simulink model "PV_GFL_864_SystemLevel_SM_R2"  (R2026a)
settings: Solver=ode23t  StopTime=0.20  MaxStep=1e-5
InitFcn:
  | run(fullfile(fileparts(get_param(bdroot,'FileName')),'..','scripts','init_pv_gfl_864_average_sm.m'));
undefined symbols (not defined in the file): Control, DiscIntNeverNeededParam, ee, GridTransformer, S1, SM, Ts
libraries: ee_lib x17, nesl_utility x15, fl_lib x5, simulink x1, eeSmAC1C x1
Description:
  | B2 readable SRF-PLL, dq measurement, and P/Q estimation on the validated B1 switching plant.
settings Model: Creator=fakebob2004  LastModifiedBy=fakebob2004

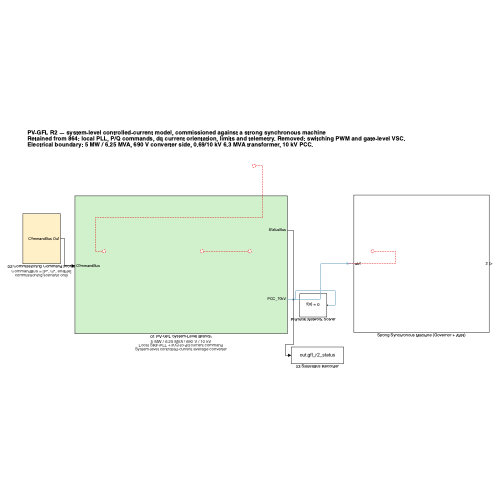
[thumbnail: Simulink's stored preview of the top-level diagram]
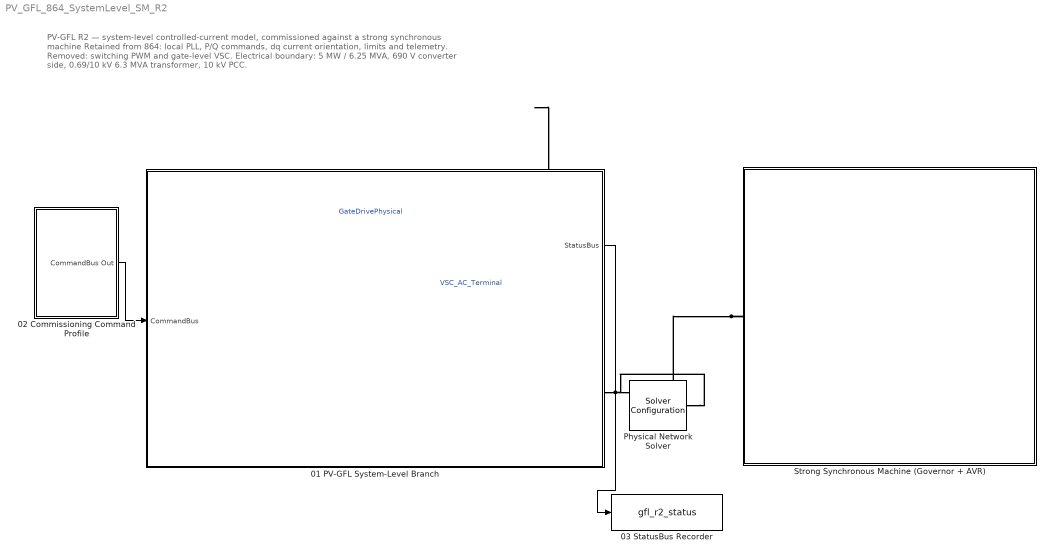
== system PV_GFL_864_SystemLevel_SM_R2 ==
  note: PV-GFL R2 — system-level controlled-current model, commissioned against a strong synchronous machine
      | Retained from 864: local PLL, P/Q commands, dq current orientation, limits and telemetry. Removed: switching PWM and gate-level VSC.
      | Electrical boundary: 5 MW / 6.25 MVA, 690 V converter side, 0.69/10 kV 6.3 MVA transformer, 10 kV PCC.
  01 PV-GFL System-Level Branch : Subsystem
      settings: AttributesFormatString=|
      | 5 MW / 6.25 MVA | 690 V / 10 kV
      | Local SRF-PLL + P/Q-to-dq current command
      | System-level controlled-current average converter
  02 Commissioning Command Profile : Subsystem
      settings: AttributesFormatString=|
      | CommandBus = [P*, Q*, enable]
      | commissioning scenario only
  03 StatusBus Recorder : ToWorkspace  VariableName=gfl_r2_status  SampleTime=-1
  Physical Network Solver : nesl_utility/Solver Configuration  PhysicalDomain=network_engine_domain  SubClassName=solver  LeftPortType=input  RightPortType=generic  Tones=[]  Harmonics=[]  SimulateNoise=off  Profile=off  UseLocalSampling=off  EnableSwitchedLinearOptims=on  FrequencyDomain=off  UseCCode=off  RelTol=0.001  AbsTol=0.001  MinStep=1e-09  ToWorkspace=off  RevertToSquareIcSolve=off  NumHomotopyIterations=100  PhasorMode=off  PhasorModeNumHarmonics=1  ConsistencySolver=NEWTON_XTOL_AFTER_FTOL  CanonicalOrdering=CANONICAL  OptimizeIntermediates=OPTIMIZED  IndexReductionMethod=DerivativeReplacement  DoDC=off  ResidualTolerance=1e-09  ConsistencyTolSource=GLOBAL  ConsistencyAbsTol=0.001  ConsistencyRelTol=0.001  ConsistencyTolFactor=0.001  UseLocalSolver=off  LocalSolverChoice=NE_BACKWARD_EULER_ADVANCER  ResolveIndetEquations=on  FunctionEvalNumThread=1  LocalSolverSampleTime=0.001  DoFixedCost=off  MaxNonlinIter=3  MaxModeIter=2  ComputeImpulses=off  ImpulseIterations=2  LinearAlgebra=auto  LinearAlgebraNumThread=0  EquationFormulation=NE_TIME_EF  DelaysMemoryBudget=1024  AutomaticFiltering=on  FilteringTimeConstant=0.001  PartitionStorageMethod=AS_NEEDED  PartitionMemoryBudget=1024  PartitionMethod=ROBUST  MultibodyUseLocalSolver=off  MultibodyLocalSolverChoice=ODE1  MultibodyLocalSolverSampleTime=0.001
  Strong Synchronous Machine (Governor + AVR) : Subsystem  VariantControl=SynchronousMachine
  wires:
  02 Commissioning Command Profile/1(CommandBus Out) -> 01 PV-GFL System-Level Branch/1(CommandBus)
  01 PV-GFL System-Level Branch/1(StatusBus) -> 03 StatusBus Recorder/1
  connections:
  ?  "VSC_AC_Terminal"
  ?  "GateDrivePhysical"
  Strong Synchronous Machine (Governor + AVR)/RConn1 -- 01 PV-GFL System-Level Branch/RConn1 -- Physical Network Solver/RConn1

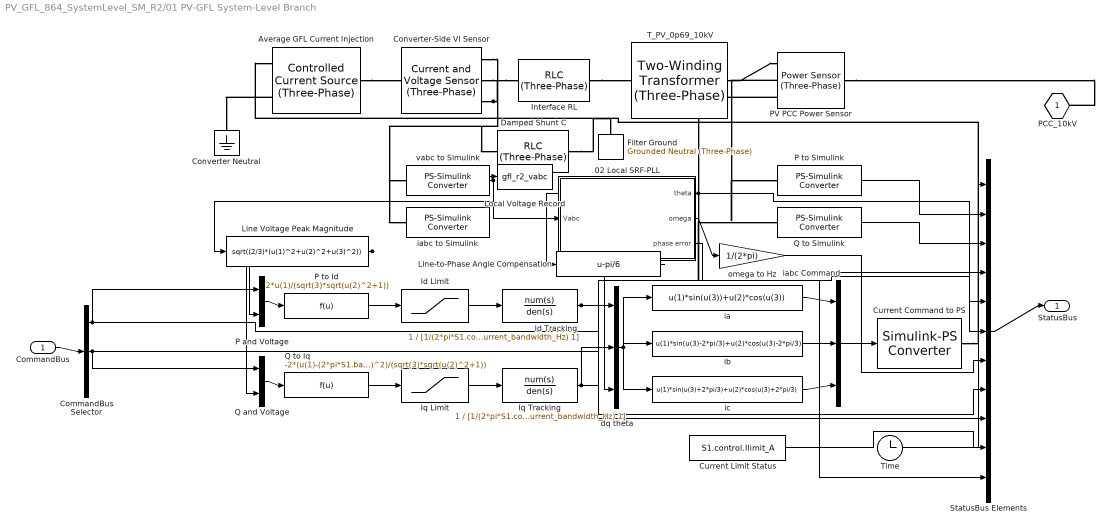
== system PV_GFL_864_SystemLevel_SM_R2/01 PV-GFL System-Level Branch ==
  CommandBus : Inport
  02 Local SRF-PLL : Subsystem
      settings: AttributesFormatString=|
      | local abc voltage only
      | wrapped phase-error PI
  Average GFL Current Injection : ee_lib/Sources/Controlled Current Source (Three-Phase)  port_option=ee.enum.threePhasePort.composite  input_option=ee.enum.inputType.instantaneous  FRated=S1.base.f_Hz Hz  G_parasitic=0 1/Ohm
  CommandBus Selector : Demux  Outputs=3
  Converter Neutral : fl_lib/Electrical/Electrical Elements/Electrical Reference
  Converter-Side VI Sensor : ee_lib/Sensors & Transducers/Current and Voltage Sensor (Three-Phase)  port_option=ee.enum.threePhasePort.composite  vMeasurementType=ee.enum.vmeasurement.ll  outputUnit=ee.enum.unit.si  SRated=100e6 A*V  VRated=24e3 V  I_specify=off  I_priority=None  I=[0, 0, 0] A  I_nominal_specify=off  I_nominal_value=1  I_nominal_unit=A  V_specify=off  V_priority=None  V=[0, 0, 0] V  V_nominal_specify=off  V_nominal_value=1  V_nominal_unit=V
  Current Command to PS : nesl_utility/Simulink-PS Converter  PhysicalDomain=network_engine_domain  SubClassName=ps_input  LeftPortType=input  RightPortType=output  PseudoPeriodic=off  Frequencies=[]  NoiseDistribution=none  NoiseParameters=[]  Unit=A  AffineConversion=off  FilteringAndDerivatives=zero  SimscapeFilterOrder=1  InputFilterTimeConstant=0.001  UdotUserProvided=0
  Current Limit Status : Constant  Value=S1.control.Ilimit_A
  Damped Shunt C : ee_lib/Passive/RLC Assemblies/RLC (Three-Phase)  port_option=ee.enum.threePhasePort.composite  component_structure=ee.enum.rlc.structure.SeriesRC  R=S1.filter.Rd_ohm Ohm  L=1e-3 H  C=S1.filter.C_F F  R_parasitic=0 Ohm  G_parasitic=0 1/Ohm  IL_specify=off  IL_priority=High  IL=[0, 0, 0] A  IL_nominal_specify=off  IL_nominal_value=1  IL_nominal_unit=A  VC_specify=off  VC_priority=High  VC=[0, 0, 0] V  VC_nominal_specify=off  VC_nominal_value=1  VC_nominal_unit=V
  Filter Ground : ee_lib/Connectors & References/Grounded Neutral (Three-Phase)  port_option=ee.enum.threePhasePort.composite
  Id Limit : Saturate  UpperLimit=S1.control.Ilimit_A  LowerLimit=-S1.control.Ilimit_A
  Id Tracking : TransferFcn  Numerator=1  Denominator=[1/(2*pi*S1.control.current_bandwidth_Hz) 1]
  Interface RL : ee_lib/Passive/RLC Assemblies/RLC (Three-Phase)  port_option=ee.enum.threePhasePort.composite  component_structure=ee.enum.rlc.structure.R  R=S1.filter.R1_ohm+S1.filter.R2_ohm Ohm  L=1e-3 H  C=1e-6 F  R_parasitic=0 Ohm  G_parasitic=0 1/Ohm  IL_specify=off  IL_priority=High  IL=[0, 0, 0] A  IL_nominal_specify=off  IL_nominal_value=1  IL_nominal_unit=A  VC_specify=off  VC_priority=High  VC=[0, 0, 0] V  VC_nominal_specify=off  VC_nominal_value=1  VC_nominal_unit=V
  Iq Limit : Saturate  UpperLimit=S1.control.Ilimit_A  LowerLimit=-S1.control.Ilimit_A
  Iq Tracking : TransferFcn  Numerator=1  Denominator=[1/(2*pi*S1.control.current_bandwidth_Hz) 1]
  Line Voltage Peak Magnitude : Fcn  Expr=sqrt((2/3)*(u(1)^2+u(2)^2+u(3)^2))
  Line-to-Phase Angle Compensation : Fcn  Expr=u-pi/6
  Local Voltage Record : ToWorkspace  VariableName=gfl_r2_vabc  SampleTime=-1
  P and Voltage : Mux  Inputs=2
  P to Id : Fcn  Expr=2*u(1)/(sqrt(3)*sqrt(u(2)^2+1))
  P to Simulink : nesl_utility/PS-Simulink Converter  PhysicalDomain=network_engine_domain  SubClassName=ps_output  LeftPortType=input  RightPortType=output  PseudoPeriodic=off  Frequencies=[]  VectorFormat=inherit  Unit=W  AffineConversion=off
  PV PCC Power Sensor : ee_lib/Sensors & Transducers/Power Sensor (Three-Phase)  port_option=ee.enum.threePhasePort.composite  load_type=ee.enum.passive.type_balanced.balanced  f0=60 Hz
  Q and Voltage : Mux  Inputs=2
  Q to Iq : Fcn  Expr=-2*(u(1)-(2*pi*S1.base.f_Hz*S1.filter.C_F/2)*u(2)^2)/(sqrt(3)*sqrt(u(2)^2+1))
  Q to Simulink : nesl_utility/PS-Simulink Converter  PhysicalDomain=network_engine_domain  SubClassName=ps_output  LeftPortType=input  RightPortType=output  PseudoPeriodic=off  Frequencies=[]  VectorFormat=inherit  Unit=W  AffineConversion=off
  StatusBus Elements : Mux  Inputs=11
  T_PV_0p69_10kV : ee_lib/Passive/Transformers/Two-Winding Transformer (Three-Phase)  SRated=S1.transformer.S_VA A*V  FRated=S1.base.f_Hz Hz  Winding1Connection=ee.enum.windingconnection.Yg  VRated1=S1.pv.Vll_low_V V  Winding2Connection=ee.enum.windingconnection.Yg  VRated2=S1.pv.Vll_high_V V  CoreType=ee.enum.coretype.threelimb  pu_Rw1=S1.transformer.R_pu/2  pu_Rw2=S1.transformer.R_pu/2  leakage_reactance_option=ee.enum.transformer_leakage.exclude  pu_Xl1=0.05  pu_Xl2=0.05  magnetizing_resistance_option=ee.enum.transformer_magnetizingResistance.exclude  pu_Rm=500  magnetizing_reactance_option=ee.enum.transformer_magnetizingReactance.exclude  saturation_option=ee.enum.transformer_saturation.exclude  pu_Xm=500  current_data=[0, .002, 1, 2]  magnetic_flux_data=[0, 1.2, 1.5, 1.51]  pu_X0=0.5  i1_specify=off  i1_priority=None  i1=[0, 0, 0] A  i1_nominal_specify=off  i1_nominal_value=1  i1_nominal_unit=A  i2_specify=off  i2_priority=None  i2=[0, 0, 0] A  i2_nominal_specify=off  i2_nominal_value=1  i2_nominal_unit=A  phi_specify=off  phi_priority=None  phi=[0, 0, 0]  phi_nominal_specify=off  phi_nominal_value=1  phi_nominal_unit=1
  Time : Clock
  dq theta : Mux  Inputs=3
  ia : Fcn  Expr=u(1)*sin(u(3))+u(2)*cos(u(3))
  iabc Command : Mux  Inputs=3
  iabc to Simulink : nesl_utility/PS-Simulink Converter  PhysicalDomain=network_engine_domain  SubClassName=ps_output  LeftPortType=input  RightPortType=output  PseudoPeriodic=off  Frequencies=[]  VectorFormat=inherit  Unit=A  AffineConversion=off
  ib : Fcn  Expr=u(1)*sin(u(3)-2*pi/3)+u(2)*cos(u(3)-2*pi/3)
  ic : Fcn  Expr=u(1)*sin(u(3)+2*pi/3)+u(2)*cos(u(3)+2*pi/3)
  omega to Hz : Gain  Gain=1/(2*pi)
  vabc to Simulink : nesl_utility/PS-Simulink Converter  PhysicalDomain=network_engine_domain  SubClassName=ps_output  LeftPortType=input  RightPortType=output  PseudoPeriodic=off  Frequencies=[]  VectorFormat=inherit  Unit=V  AffineConversion=off
  PCC_10kV : PMIOPort  Side=Right  ConnectionType=Connection: foundation.electrical.three_phase
  StatusBus : Outport
  wires:
  CommandBus/1 -> CommandBus Selector/1
  vabc to Simulink/1 -> Local Voltage Record/1, 02 Local SRF-PLL/1(Vabc), Line Voltage Peak Magnitude/1
  CommandBus Selector/1 -> P and Voltage/1, StatusBus Elements/4
  Line Voltage Peak Magnitude/1 -> P and Voltage/2, Q and Voltage/2
  CommandBus Selector/2 -> Q and Voltage/1, StatusBus Elements/5
  P and Voltage/1 -> P to Id/1
  P to Id/1 -> Id Limit/1
  Id Limit/1 -> Id Tracking/1
  Q and Voltage/1 -> Q to Iq/1
  Q to Iq/1 -> Iq Limit/1
  Iq Limit/1 -> Iq Tracking/1
  Id Tracking/1 -> dq theta/1, StatusBus Elements/8
  Iq Tracking/1 -> dq theta/2, StatusBus Elements/9
  02 Local SRF-PLL/1(theta) -> Line-to-Phase Angle Compensation/1, StatusBus Elements/6
  Line-to-Phase Angle Compensation/1 -> dq theta/3
  dq theta/1 -> ia/1, ib/1, ic/1
  ia/1 -> iabc Command/1
  ib/1 -> iabc Command/2
  ic/1 -> iabc Command/3
  iabc Command/1 -> Current Command to PS/1
  02 Local SRF-PLL/2(omega) -> omega to Hz/1
  Time/1 -> StatusBus Elements/1
  P to Simulink/1 -> StatusBus Elements/2
  Q to Simulink/1 -> StatusBus Elements/3
  omega to Hz/1 -> StatusBus Elements/7
  Current Limit Status/1 -> StatusBus Elements/10
  02 Local SRF-PLL/3(phase error) -> StatusBus Elements/11
  StatusBus Elements/1 -> StatusBus/1
  connections:
  Average GFL Current Injection/LConn2 -- Converter Neutral/LConn1
  Average GFL Current Injection/RConn1 -- Converter-Side VI Sensor/LConn1
  Interface RL/LConn1 -- Converter-Side VI Sensor/RConn3 -- Damped Shunt C/LConn1
  Damped Shunt C/RConn1 -- Filter Ground/LConn1
  Interface RL/RConn1 -- T_PV_0p69_10kV/LConn1
  T_PV_0p69_10kV/RConn1 -- PV PCC Power Sensor/LConn1
  PV PCC Power Sensor/RConn1 -- PCC_10kV/RConn1
  Converter-Side VI Sensor/RConn1 -- vabc to Simulink/LConn1
  Converter-Side VI Sensor/RConn2 -- iabc to Simulink/LConn1
  PV PCC Power Sensor/LConn2 -- P to Simulink/LConn1
  PV PCC Power Sensor/LConn3 -- Q to Simulink/LConn1
  Current Command to PS/RConn1 -- Average GFL Current Injection/LConn1

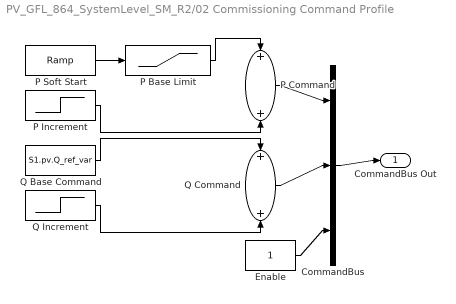
== system PV_GFL_864_SystemLevel_SM_R2/02 Commissioning Command Profile ==
  CommandBus : Mux  Inputs=3
  Enable : Constant
  P Base Limit : Saturate  UpperLimit=S1.pv.P_initial_W  LowerLimit=0
  P Command : Sum
  P Increment : Step  Time=S1.pv.P_step_time_s  FinalValue=S1.pv.P_final_W-S1.pv.P_initial_W  SampleTime=0
  P Soft Start : simulink/Sources/Ramp  slope=S1.pv.P_ramp_W_per_s  start=0  InitialOutput=0
  Q Base Command : Constant  Value=S1.pv.Q_ref_var
  Q Command : Sum
  Q Increment : Step  Time=S1.pv.Q_step_time_s  FinalValue=S1.pv.Q_step_var  SampleTime=0
  CommandBus Out : Outport
  wires:
  P Soft Start/1 -> P Base Limit/1
  P Base Limit/1 -> P Command/1
  P Increment/1 -> P Command/2
  Q Base Command/1 -> Q Command/1
  Q Increment/1 -> Q Command/2
  P Command/1 -> CommandBus/1
  Q Command/1 -> CommandBus/2
  Enable/1 -> CommandBus/3
  CommandBus/1 -> CommandBus Out/1

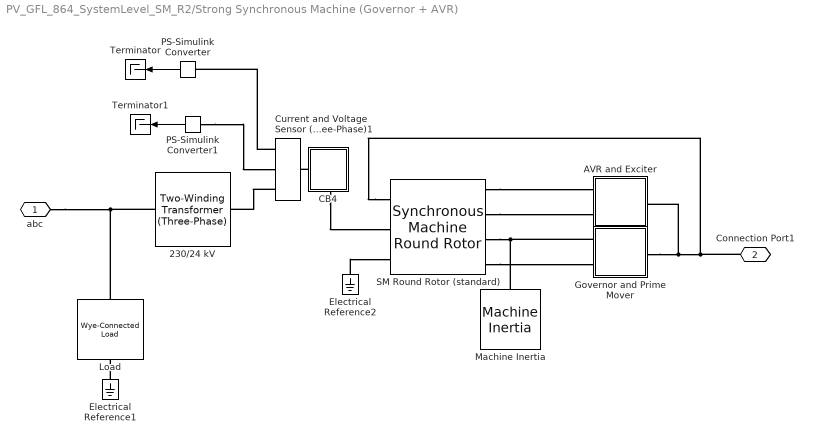
== system PV_GFL_864_SystemLevel_SM_R2/Strong Synchronous Machine (Governor + AVR) ==
  " Load" : ee_lib/Passive/RLC Assemblies/Wye-Connected Load  port_option=ee.enum.threePhasePort.composite  parameterization=ee.enum.rlc.parameterization.ratedpower  component_structure=ee.enum.rlc.structure.R  component_structure_PQ=ee.enum.rlc.structure.ParallelRL  R=1 Ohm  L=1e-3 H  C=1e-6 F  VRated=Grid.voltage V  FRated=Grid.frequency Hz  P=SM.P_load W  Qpos=SM.Q_load A*V  Qneg=-1e2 A*V  R_parasitic=0 Ohm  G_parasitic=0 1/Ohm  R_parasitic_PQ=0 Ohm  G_parasitic_PQ=0 1/Ohm  Vmag0=4.16e3 V  Vang0=0 deg  Freq0=60 Hz  IL_specify=off  IL_priority=High  IL=[0, 0, 0] A  IL_nominal_specify=off  IL_nominal_value=1  IL_nominal_unit=A  VC_specify=off  VC_priority=High  VC=[0, 0, 0] V  VC_nominal_specify=off  VC_nominal_value=1  VC_nominal_unit=V
  230/24 kV : ee_lib/Passive/Transformers/Two-Winding Transformer (Three-Phase)  SRated=SM.MVA V*A  FRated=Grid.frequency Hz  Winding1Connection=ee.enum.windingconnection.delta1  VRated1=Grid.voltage V  Winding2Connection=ee.enum.windingconnection.delta11  VRated2=SM.Voltage V  CoreType=ee.enum.coretype.fivelimb  pu_Rw1=GridTransformer.winding_resistance/2  pu_Rw2=GridTransformer.winding_resistance/2  leakage_reactance_option=ee.enum.transformer_leakage.include  pu_Xl1=GridTransformer.winding_lekage_reactance/2  pu_Xl2=GridTransformer.winding_lekage_reactance/2  magnetizing_resistance_option=ee.enum.transformer_magnetizingResistance.exclude  pu_Rm=500  magnetizing_reactance_option=ee.enum.transformer_magnetizingReactance.include  saturation_option=ee.enum.transformer_saturation.exclude  pu_Xm=500  current_data=[0, .002, 1, 2]  magnetic_flux_data=[0, 1.2, 1.5, 1.51]  pu_X0=0.0586/2  i1_specify=off  i1_priority=None  i1=[ 0 0 0 ] A  i1_nominal_specify=off  i1_nominal_value=1  i1_nominal_unit=A  i2_specify=off  i2_priority=None  i2=[ 0 0 0 ] A  i2_nominal_specify=off  i2_nominal_value=1  i2_nominal_unit=A  phi_specify=off  phi_priority=None  phi=[ 0 0 0 ]  phi_nominal_specify=off  phi_nominal_value=1  phi_nominal_unit=1
  AVR and Exciter : Subsystem
  CB4 : Subsystem
      settings: PortSchema="{\"entries\":[{\"content\":{\"sides\":[{\"content\":{\"connectorIds\":[\"LConn1\"]},\"type\":\"ConnectorPlacement.EquallySpacedRectSide\",\"uuid\":\"24022911-97b6-486c-a625-f0780a134feb\"},{\"content\":{\"connectorIds\":[],\"side\":\"RIGHT\"},\"type\":\"ConnectorPlacement.EquallySpacedRectSide\",\"uuid\":\"1242aa8b-343b-4af2-8b96-dfa58505a53d\"},{\"content\":{\"connectorIds\":[],\"side\":\"TOP\"},\"type\":\"ConnectorPlacement.EquallySpacedRectSide\",\"uuid\":\"e73be2e9-5300-480f-914f-665ff518f6ad\"},{\"content\":{\"connectorIds\":[\"RConn1\"],\"side\":\"BOTTOM\"},\"type\":\"ConnectorPlacement.EquallySpacedRectSide\",\"uuid\":\"6525202c-c4e7-4c96-9421-427b801d0594\"}]},\"type\":\"ConnectorPlacement.EquallySpacedConnector\",\"uuid\":\"b455682c-e951-4ef6-bff8-cd3f50b315f1\"}],\"packageUris\":[\"http://schema.mathworks.com/mf0/Connector/R2020b\"],\"version\":\"1.0\"}"
      mask Display: image('$imagefile'); % Use "Edit Image" on toolstrip to change.
  Current and Voltage Sensor (Three-Phase)1 : ee_lib/Sensors & Transducers/Current and Voltage Sensor (Three-Phase)  port_option=ee.enum.threePhasePort.composite  vMeasurementType=ee.enum.vmeasurement.ll  outputUnit=ee.enum.unit.pu  SRated=100e6 A*V  VRated=4.16e3 V  I_specify=off  I_priority=None  I=[0, 0, 0] A  I_nominal_specify=off  I_nominal_value=1  I_nominal_unit=A  V_specify=off  V_priority=None  V=[0, 0, 0] V  V_nominal_specify=off  V_nominal_value=1  V_nominal_unit=V
  Electrical Reference1 : fl_lib/Electrical/Electrical Elements/Electrical Reference
  Electrical Reference2 : fl_lib/Electrical/Electrical Elements/Electrical Reference
  "Governor and Prime Mover " : Subsystem  mask(Governor and Prime Mover){pu_speed_reference=SM.speed_reference, droop_percentage=SM.droop_p, pu_load_reference_setpoint=SM.load_reference_set_point, T_G=SM.governor_time_constant, T_CH=SM.time_constsnt_steamchest, base_torque=SM.Base_Torque_SM, pu_torque0=SM.initial_torque}
      mask prompts: pu_speed_reference "Speed reference, (pu)"; droop_percentage "Percentage droop, (%)"; pu_load_reference_setpoint "Load reference setpoint, (pu)"; T_G "Time constant of governor, (s)"; T_CH "Time constant of main inlet volumes and steam chest, (s)"; base_torque "Base torque, (N*m)"; pu_torque0 "Initial torque, (pu)"
      mask help:
      | Implements a synchronous machine governor and prime mover. The prime mover is a non-reheat steam turbine.
      |
      | The input to the block is a per-unit synchronous machine measurement vector.
      |
      | R and C are mechanical rotational ports.
  Machine Inertia : ee_lib/Electromechanical/Mechanical/Machine Inertia  SRated=SM.MVA V*A  FRated=Grid.frequency Hz  nPolePairs=SM.polepairs  inertia_option=2  J=27548 kg*m^2  H=SM.inertia s  damper_option=2  D=39.0509 N*m/(rad/s)  pu_D=SM.damping  initialization_option=2  fMechanical0=60 Hz  fElectrical0=Grid.frequency Hz
  PS-Simulink Converter : nesl_utility/PS-Simulink Converter  PhysicalDomain=network_engine_domain  SubClassName=ps_output  LeftPortType=input  RightPortType=output  PseudoPeriodic=off  Frequencies=[]  VectorFormat=inherit  Unit=inherit  AffineConversion=off
  PS-Simulink Converter1 : nesl_utility/PS-Simulink Converter  PhysicalDomain=network_engine_domain  SubClassName=ps_output  LeftPortType=input  RightPortType=output  PseudoPeriodic=off  Frequencies=[]  VectorFormat=inherit  Unit=inherit  AffineConversion=off
  SM Round Rotor (standard) : ee_lib/Electromechanical/Synchronous/Synchronous Machine Round Rotor  port_option=ee.enum.threePhasePort.composite  SRated=SM.MVA V*A  VRated=SM.Voltage V  FRated=Grid.frequency Hz  nPolePairs=SM.polepairs  param_option=ee.enum.sm.parameterization.standard  fieldCircuitParameterization_option=2  baseEfd=92.95 V  baseIfd=SM.field_current A  zero_sequence=ee.enum.park.zerosequence.include  axes_param=ee.enum.rotorangle.qaxis  Ladu=1.66  Laqu=1.61  L0=0.15  Ll=0.15  Ra=SM.stator_resistance  Lfd=0.165  Rfd=0.0006  L1d=0.1713  R1d=0.0284  L1q=0.7252  R1q=0.00619  L2q=0.125  R2q=0.02368  Xl=SM.lekage_reactance  Xd=SM.xd  Xq=SM.xq  X0=0.15  Xdd=SM.xd_  Xqd=SM.xq_  Xddd=SM.xd_dash  Xqdd=SM.xq_dash  d_option=1  Td0d=SM.Tdo_ s  Tdd=1.3260 s  Td0dd=SM.Tdo_dash s  Tddd=0.0230 s  q_option=1  Tq0d=SM.Tqo_ s  Tqd=0.3693 s  Tq0dd=SM.Tqo_dash s  Tqdd=0.0269 s  saturation_option=0  saturation_ifd=[0.00, 0.48, 0.76, 1.38, 1.79]  saturation_Vag=[0.00, 0.80, 1.08, 1.31, 1.40]  initialization_option=2  source_type=ee.enum.sm.load_flow_source_type.Swing  Vmag0=SM.Voltage V  Vang0=0 deg  Pt0=SM.initial_Pe V*A  Qt0=SM.initial_Qe V*A  minimum_pu=0.95  phase_search_range=[-inf, inf] deg  gmin=1e-6 S  connection_option=int32(ee.enum.Connection.wye)  num_q_dampers=2  rotor_offset=-pi / 2 rad  pu_psid_specify=on  pu_psid_priority=High  pu_psid=0  pu_psid_nominal_specify=off  pu_psid_nominal_value=1  pu_psid_nominal_unit=1  pu_psiq_specify=on  pu_psiq_priority=High  pu_psiq=0  pu_psiq_nominal_specify=off  pu_psiq_nominal_value=1  pu_psiq_nominal_unit=1  pu_psifd_specify=on  pu_psifd_priority=High  pu_psifd=0  pu_psifd_nominal_specify=off  pu_psifd_nominal_value=1  pu_psifd_nominal_unit=1  pu_psi1d_specify=on  pu_psi1d_priority=High  pu_psi1d=0  pu_psi1d_nominal_specify=off  pu_psi1d_nominal_value=1  pu_psi1d_nominal_unit=1  pu_psi1q_specify=on  pu_psi1q_priority=High  pu_psi1q=0  pu_psi1q_nominal_specify=off  pu_psi1q_nominal_value=1  pu_psi1q_nominal_unit=1  pu_psi2q_specify=on  pu_psi2q_priority=High  pu_psi2q=0  pu_psi2q_nominal_specify=off  pu_psi2q_nominal_value=1  pu_psi2q_nominal_unit=1  angular_position_diff_specify=on  angular_position_diff_priority=High  angular_position_diff=0 deg  angular_position_diff_nominal_specify=off  angular_position_diff_nominal_value=1  angular_position_diff_nominal_unit=deg  Tmeas=298.15 K  alpha=3.93e-3 1/K  stator_thermal_mass=100 J/K  rotor_thermal_mass=200 J/K  temperatureA_specify=off  temperatureA_priority=High  temperatureA=25 degC  temperatureA_nominal_specify=off  temperatureA_nominal_value=1  temperatureA_nominal_unit=degC  temperatureB_specify=off  temperatureB_priority=High  temperatureB=25 degC  temperatureB_nominal_specify=off  temperatureB_nominal_value=1  temperatureB_nominal_unit=degC  temperatureC_specify=off  temperatureC_priority=High  temperatureC=25 degC  temperatureC_nominal_specify=off  temperatureC_nominal_value=1  temperatureC_nominal_unit=degC  temperatureR_specify=off  temperatureR_priority=High  temperatureR=25 degC  temperatureR_nominal_specify=off  temperatureR_nominal_value=1  temperatureR_nominal_unit=degC
  Terminator : Terminator
  Terminator1 : Terminator
  abc : PMIOPort  Side=Right
  Connection Port1 : PMIOPort  Port=2  Side=Left
  wires:
  PS-Simulink Converter1/1 -> Terminator1/1
  PS-Simulink Converter/1 -> Terminator/1
  connections:
  Electrical Reference2/LConn1 -- SM Round Rotor (standard)/RConn3
  CB4/RConn1 -- SM Round Rotor (standard)/RConn2
  PS-Simulink Converter1/LConn1 -- Current and Voltage Sensor (Three-Phase)1/RConn2
  Current and Voltage Sensor (Three-Phase)1/RConn3 -- 230/24 kV/RConn1
  SM Round Rotor (standard)/LConn2 -- AVR and Exciter/RConn2
  Electrical Reference1/LConn1 -- " Load"/RConn1
  CB4/LConn1 -- Current and Voltage Sensor (Three-Phase)1/LConn1
  SM Round Rotor (standard)/LConn1 -- AVR and Exciter/RConn1
  Current and Voltage Sensor (Three-Phase)1/RConn1 -- PS-Simulink Converter/LConn1
  SM Round Rotor (standard)/LConn4 -- "Governor and Prime Mover "/RConn2
  "Governor and Prime Mover "/RConn1 -- Machine Inertia/LConn1 -- SM Round Rotor (standard)/LConn3
  SM Round Rotor (standard)/RConn1 -- Connection Port1/RConn1 -- AVR and Exciter/LConn1 -- "Governor and Prime Mover "/LConn1
  230/24 kV/LConn1 -- abc/RConn1 -- " Load"/LConn1

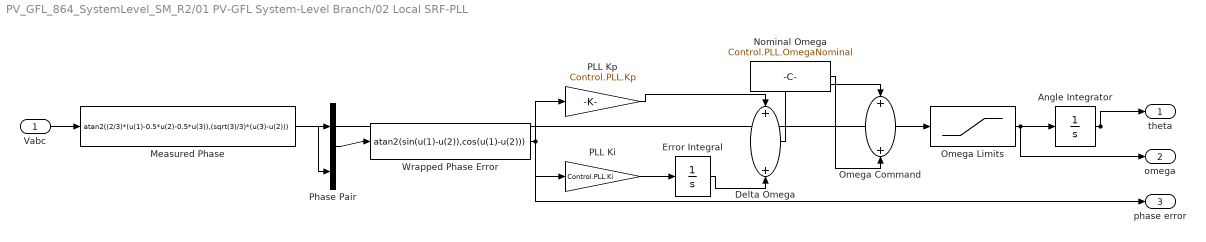
== system PV_GFL_864_SystemLevel_SM_R2/01 PV-GFL System-Level Branch/02 Local SRF-PLL ==
  Vabc : Inport
  Angle Integrator : Integrator  InitialCondition=Control.PLL.Theta0
  Delta Omega : Sum
  Error Integral : Integrator
  Measured Phase : Fcn  Expr=atan2((2/3)*(u(1)-0.5*u(2)-0.5*u(3)),(sqrt(3)/3)*(u(3)-u(2)))
  Nominal Omega : Constant  Value=Control.PLL.OmegaNominal
  Omega Command : Sum
  Omega Limits : Saturate  UpperLimit=Control.PLL.OmegaMax  LowerLimit=Control.PLL.OmegaMin
  PLL Ki : Gain  Gain=Control.PLL.Ki
  PLL Kp : Gain  Gain=Control.PLL.Kp
  Phase Pair : Mux  Inputs=2
  Wrapped Phase Error : Fcn  Expr=atan2(sin(u(1)-u(2)),cos(u(1)-u(2)))
  theta : Outport
  omega : Outport  Port=2
  phase error : Outport  Port=3
  wires:
  Vabc/1 -> Measured Phase/1
  Measured Phase/1 -> Phase Pair/1
  Angle Integrator/1 -> Phase Pair/2, theta/1
  Phase Pair/1 -> Wrapped Phase Error/1
  Wrapped Phase Error/1 -> PLL Kp/1, PLL Ki/1, phase error/1
  PLL Ki/1 -> Error Integral/1
  PLL Kp/1 -> Delta Omega/1
  Error Integral/1 -> Delta Omega/2
  Delta Omega/1 -> Omega Command/1
  Nominal Omega/1 -> Omega Command/2
  Omega Command/1 -> Omega Limits/1
  Omega Limits/1 -> Angle Integrator/1, omega/1

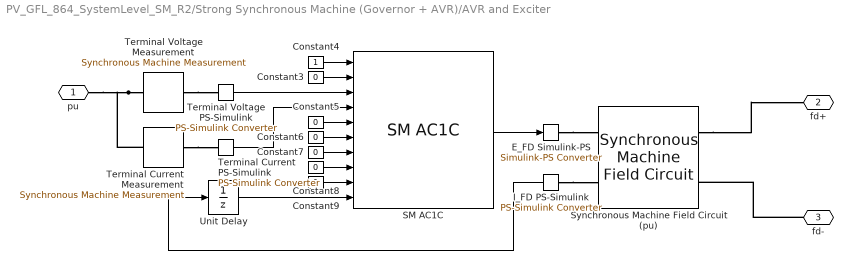
== system PV_GFL_864_SystemLevel_SM_R2/Strong Synchronous Machine (Governor + AVR)/AVR and Exciter ==
  Constant{3,5..9} (6 alike) : Constant  Value=0
  Constant4 : Constant
  "E_FD Simulink-PS " : nesl_utility/Simulink-PS Converter  PhysicalDomain=network_engine_domain  SubClassName=ps_input  LeftPortType=input  RightPortType=output  PseudoPeriodic=off  Frequencies=[]  NoiseDistribution=none  NoiseParameters=[]  Unit=1  AffineConversion=off  FilteringAndDerivatives=zero  SimscapeFilterOrder=1  InputFilterTimeConstant=.001  UdotUserProvided=0
  I_FD PS-Simulink : nesl_utility/PS-Simulink Converter  PhysicalDomain=network_engine_domain  SubClassName=ps_output  LeftPortType=input  RightPortType=output  PseudoPeriodic=off  Frequencies=[]  VectorFormat=1-D array  Unit=1  AffineConversion=off
  SM AC1C : eeSmAC1C/SM AC1C  E_FD0=1  Ts=-1  R_C=0  X_C=0  T_R=0  K_A=600  T_A=0.01  T_B=0  T_C=0  K_F=0.35  T_F=0.5  V_Amax=14.5  V_Amin=-14.5  E_FEmax=6.03  E_FEmin=-5.43  oelInputLocation=Unused  uelInputLocation=Unused  sclInputLocation=Unused  K_E=1  T_E=0.08  K_C=0.2  K_D=0.38  E_1=4.18  S_E_E1=0.1  E_2=3.14  S_E_E2=0.03  V_FEmax=99  V_Emin=0
  Synchronous Machine Field Circuit (pu) : ee_lib/Electromechanical/Synchronous/Synchronous Machine Field Circuit  unit_option=ee.enum.unit.pu  SRated=SM.MVA V*A  FRated=60 Hz  fieldCircuitParameterization_option=2  baseEfd=92.95 V  baseIfd=1300 A  parameterization_option=2  Ladu=1.66  Rfd=0.0006  Xl=SM.lekage_reactance  Xd=SM.xd  Xdd=SM.xd_  Xddd=SM.xd_dash  d_option=ee.enum.circuit.open  Td0d=SM.Tdo_ s  Tdd=1.3260 s  Td0dd=SM.Tdo_dash s  Tddd=0.0230 s
  Terminal Current Measurement : ee_lib/Electromechanical/Synchronous/Synchronous Machine Measurement  output_idx=15
  Terminal Current PS-Simulink : nesl_utility/PS-Simulink Converter  PhysicalDomain=network_engine_domain  SubClassName=ps_output  LeftPortType=input  RightPortType=output  PseudoPeriodic=off  Frequencies=[]  VectorFormat=1-D array  Unit=1  AffineConversion=off
  Terminal Voltage Measurement : ee_lib/Electromechanical/Synchronous/Synchronous Machine Measurement  output_idx=14
  Terminal Voltage PS-Simulink : nesl_utility/PS-Simulink Converter  PhysicalDomain=network_engine_domain  SubClassName=ps_output  LeftPortType=input  RightPortType=output  PseudoPeriodic=off  Frequencies=[]  VectorFormat=1-D array  Unit=1  AffineConversion=off
  Unit Delay : UnitDelay  InitialCondition=1.32943  SampleTime=-1
  pu : PMIOPort  Side=Left
  fd+ : PMIOPort  Port=2  Side=Right
  fd- : PMIOPort  Port=3  Side=Right
  wires:
  I_FD PS-Simulink/1 -> Unit Delay/1
  Terminal Voltage PS-Simulink/1 -> SM AC1C/3
  Constant3/1 -> SM AC1C/2
  Constant4/1 -> SM AC1C/1
  Constant5/1 -> SM AC1C/5
  Constant6/1 -> SM AC1C/6
  Constant7/1 -> SM AC1C/7
  Constant8/1 -> SM AC1C/8
  Constant9/1 -> SM AC1C/9
  Unit Delay/1 -> SM AC1C/10
  SM AC1C/1 -> "E_FD Simulink-PS "/1
  Terminal Current PS-Simulink/1 -> SM AC1C/4
  connections:
  "E_FD Simulink-PS "/RConn1 -- Synchronous Machine Field Circuit (pu)/LConn1
  I_FD PS-Simulink/LConn1 -- Synchronous Machine Field Circuit (pu)/LConn2
  fd-/RConn1 -- Synchronous Machine Field Circuit (pu)/RConn2
  Synchronous Machine Field Circuit (pu)/RConn1 -- fd+/RConn1
  Terminal Voltage Measurement/LConn1 -- Terminal Current Measurement/LConn1 -- pu/RConn1
  Terminal Voltage Measurement/RConn1 -- Terminal Voltage PS-Simulink/LConn1
  Terminal Current Measurement/RConn1 -- Terminal Current PS-Simulink/LConn1

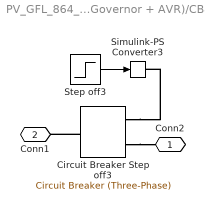
== system PV_GFL_864_SystemLevel_SM_R2/Strong Synchronous Machine (Governor + AVR)/CB4 ==
  Circuit Breaker Step off3 : ee_lib/Switches & Breakers/Circuit Breaker (Three-Phase)  port_option=ee.enum.threePhasePort.composite  control_port_option=ee.enum.controlport.ps  R_closed=0.001 Ohm  G_open=1e-4 1/Ohm  threshold=0.5 V  breaker_behavior=ee.enum.switches.breakerBehavior.zeroCrossingEnable  i_th=1e-8 A
  Simulink-PS Converter3 : nesl_utility/Simulink-PS Converter  PhysicalDomain=network_engine_domain  SubClassName=ps_input  LeftPortType=input  RightPortType=output  PseudoPeriodic=off  Frequencies=[]  NoiseDistribution=none  NoiseParameters=[]  Unit=1  AffineConversion=off  FilteringAndDerivatives=zero  SimscapeFilterOrder=1  InputFilterTimeConstant=0.001  UdotUserProvided=1
  Step off3 : Step  Time=0  FinalValue=0  SampleTime=Ts
  Conn2 : PMIOPort  Side=Left
  Conn1 : PMIOPort  Port=2  Side=Right
  wires:
  Step off3/1 -> Simulink-PS Converter3/1
  connections:
  Circuit Breaker Step off3/RConn1 -- Conn1/RConn1
  Circuit Breaker Step off3/LConn1 -- Simulink-PS Converter3/RConn1
  Circuit Breaker Step off3/LConn2 -- Conn2/RConn1

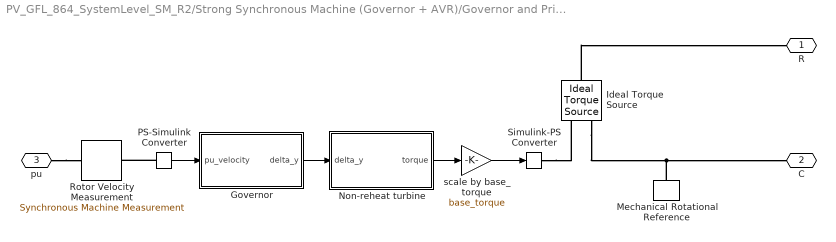
== system PV_GFL_864_SystemLevel_SM_R2/Strong Synchronous Machine (Governor + AVR)/Governor and Prime Mover  ==
  Governor : Subsystem
  Ideal Torque Source : fl_lib/Mechanical/Mechanical Sources/Ideal Torque Source
  Mechanical Rotational Reference : fl_lib/Mechanical/Rotational Elements/Mechanical Rotational Reference
  Non-reheat turbine : Subsystem
  PS-Simulink Converter : nesl_utility/PS-Simulink Converter  PhysicalDomain=network_engine_domain  SubClassName=ps_output  LeftPortType=input  RightPortType=output  PseudoPeriodic=off  Frequencies=[]  VectorFormat=1-D array  Unit=1  AffineConversion=off
  Rotor Velocity Measurement : ee_lib/Electromechanical/Synchronous/Synchronous Machine Measurement  output_idx=4
  Simulink-PS Converter : nesl_utility/Simulink-PS Converter  PhysicalDomain=network_engine_domain  SubClassName=ps_input  LeftPortType=input  RightPortType=output  PseudoPeriodic=off  Frequencies=[]  NoiseDistribution=none  NoiseParameters=[]  Unit=1  AffineConversion=off  FilteringAndDerivatives=zero  SimscapeFilterOrder=1  InputFilterTimeConstant=0.001  UdotUserProvided=1
  scale by base_torque : Gain  Gain=base_torque
  R : PMIOPort  Side=Right
  C : PMIOPort  Port=2  Side=Right
  pu : PMIOPort  Port=3  Side=Left
  wires:
  scale by base_torque/1 -> Simulink-PS Converter/1
  Non-reheat turbine/1(torque) -> scale by base_torque/1
  Governor/1(delta_y) -> Non-reheat turbine/1(delta_y)
  PS-Simulink Converter/1 -> Governor/1(pu_velocity)
  connections:
  Simulink-PS Converter/RConn1 -- Ideal Torque Source/RConn1
  PS-Simulink Converter/LConn1 -- Rotor Velocity Measurement/RConn1
  pu/RConn1 -- Rotor Velocity Measurement/LConn1
  Ideal Torque Source/LConn1 -- R/RConn1
  Mechanical Rotational Reference/LConn1 -- Ideal Torque Source/RConn2 -- C/RConn1

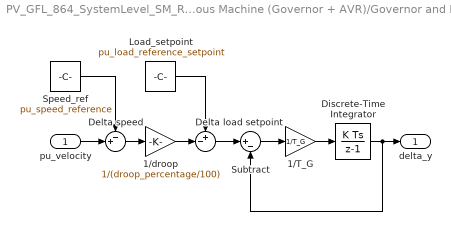
== system PV_GFL_864_SystemLevel_SM_R2/Strong Synchronous Machine (Governor + AVR)/Governor and Prime Mover /Governor ==
  pu_velocity : Inport
  1/T_G : Gain  Gain=1/T_G
  1/droop : Gain  Gain=1/(droop_percentage/100)
  Delta load setpoint : Sum  Inputs=+-|
  Delta speed : Sum  Inputs=-+|
  Discrete-Time Integrator : DiscreteIntegrator  InitialCondition=pu_torque0  SampleTime=Ts  ICPrevOutput=DiscIntNeverNeededParam  ICPrevScaledInput=DiscIntNeverNeededParam
  Load_setpoint : Constant  Value=pu_load_reference_setpoint  SampleTime=Ts
  Speed_ref : Constant  Value=pu_speed_reference  SampleTime=Ts
  Subtract : Sum  Inputs=|+-
  delta_y : Outport  VectorParamsAs1DForOutWhenUnconnected=off
  wires:
  Discrete-Time Integrator/1 -> Subtract/2, delta_y/1
  1/T_G/1 -> Discrete-Time Integrator/1
  Subtract/1 -> 1/T_G/1
  Delta load setpoint/1 -> Subtract/1
  1/droop/1 -> Delta load setpoint/2
  pu_velocity/1 -> Delta speed/2
  Load_setpoint/1 -> Delta load setpoint/1
  Delta speed/1 -> 1/droop/1
  Speed_ref/1 -> Delta speed/1

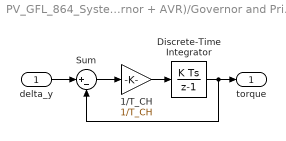
== system PV_GFL_864_SystemLevel_SM_R2/Strong Synchronous Machine (Governor + AVR)/Governor and Prime Mover /Non-reheat turbine ==
  delta_y : Inport
  1/T_CH : Gain  Gain=1/T_CH
  Discrete-Time Integrator : DiscreteIntegrator  InitialCondition=pu_torque0  SampleTime=Ts  ICPrevOutput=DiscIntNeverNeededParam  ICPrevScaledInput=DiscIntNeverNeededParam
  Sum : Sum  Inputs=|+-
  torque : Outport  VectorParamsAs1DForOutWhenUnconnected=off
  wires:
  Discrete-Time Integrator/1 -> torque/1, Sum/2
  1/T_CH/1 -> Discrete-Time Integrator/1
  Sum/1 -> 1/T_CH/1
  delta_y/1 -> Sum/1
